simulink model "single_phase_afe_ideal"  (R2026a)
settings: Solver=ode23tb  StopTime=simlength  FixedStep=tc  MaxStep=glb_time.tc
values from neighbouring files (symbols this model uses):
  afe_ctrl = ctrl_afe_setup(glb_time.ts_afe, grid_emu.omega_grid_nom)    [init_model_legacy.m]
  frequency_set = 300    [init_model_legacy.m]
  glb_time = timing_setup(fpwm_afe, trgo_afe, fpwm_inv, trgo_inv, fpwm_single_phase_inv, trgo_single_phase_inv, fpwm_dab, trgo_dab,      fpwm_psfbc, trgo_psfbc, fpwm_isop_rail, trgo_isop_rail, fpwm_cllc, trgo_cllc, t_measure, tc_factor, tc_decimation, delay_pwm, dead_time_afe,      dead_time_inv, dead_time_single_phase_inv, dead_time_dab, dead_time_psfbc, dead_time_isop_rail, dead_time_cllc)    [init_model_legacy.m]
  grid_emu = grid_three_phase_emulator('Dyn11', delta_star, grid_nominal_power, application_voltage, us1, us2, fgrid,                  eq_grid_inductance, eq_grid_resistance, eta, ucc, i1m, p_iron, n1, n2, core_area, core_length, mur,                  up_xi_pu_ref, up_eta_pu_ref, un_xi_pu_ref, un_eta_pu_ref)    [init_model_legacy.m]
  heatsink = liquid_cooled_plate_2kw_setup(weight, no_weight, cp_al, heat_capacity_hs, thermal_conductivity_al,      Rth_switch_HA, Rth_mosfet_HA, Rth_diode_HA, Tambient, DThs_init)    [init_model_legacy.m]
  kepsilon = 2    [init_model_legacy.m]
  omega_set = frequency_set*2*pi    (= 1884.95559215)    [init_model_legacy.m]
  single_phase_inverter_ctrl = ctrl_single_phase_inverter_setup(glb_time.ts_inv, pres_ctrl.omega_set,      dqvector_pi.kp_inv, dqvector_pi.ki_inv, pres_ctrl.kp_rpi, pres_ctrl.ki_rpi, pres_ctrl.delta_rpi)    [init_model_legacy.m]
  Tambient = 40    [init_model_legacy.m]
  time_step_ref_1 = 0.025    [init_model_legacy.m]
  time_step_ref_2 = 0.5    [init_model_legacy.m]
  time_step_ref_3 = 1    [init_model_legacy.m]
  Vdc_nom = 400*1.35    (= 540)    [power_losses_calculation.m]
undefined symbols (not defined in the file or in its folder): delta_fht1, hwdata, igbt, Ld_fht1, magnitude, omega_fht1, ts_inv, Vac_FS, Xbez
libraries: fl_lib x116, nesl_utility x65, phase_shift_filter_ccaller x5, dq_vector_pi x4, igbt_simple_2th_lib x4, linear_double_integrator_observer_ccaller x3, lithium_ion_battery x1, dclink_for_two_levels x1, three_phase_voltage_with_frt_emulator x1, simulink x1, cstblocks_lti x1, single_phase_pwm_modulator x1
(part 6 of 6)

== matlab function single_phase_afe_ideal/single_phase_inverter/single phase inverter control/single_phase_inverter_ctrl/dclink_ripple_compensation_rpi/dq2alphabeta/MATLAB Function ==
  data: d input; alpha output; q input; phase input; beta output
function [alpha, beta] = dq2alphabeta(d, q, phase)

alpha = d*cos(phase) - q*sin(phase);
beta = d*sin(phase) + q*cos(phase);

== matlab function single_phase_afe_ideal/single_phase_inverter/single phase inverter control/single_phase_inverter_ctrl/phase generator/FHT-PLL/pll_stageB/double_integrator_observer/bounder2 ==
  data: u input; y output
function y = bounder(u)
    
    y = -pi + mod(u+3*pi,2*pi);
    
end

== matlab function single_phase_afe_ideal/single_phase_inverter/single phase inverter control/single_phase_inverter_ctrl/dclink_ripple_compensation_dq/dq_vector_pi1/alphabeta2dq/MATLAB Function ==
  data: alpha input; d output; beta input; phase input; q output
function [d, q] = alphabeta2dq(alpha, beta, phase)

d = alpha*cos(phase) + beta*sin(phase);
q = -alpha*sin(phase) + beta*cos(phase);

== matlab function single_phase_afe_ideal/single_phase_inverter/single phase inverter control/single_phase_inverter_ctrl/phase generator/FHT-PLL/pll_stageA/filter_and_transformation/abc2alphabeta ==
  data: a input; alpha output; b input; c input; beta output
function [alpha,beta] = abc2alphabeta(a,b,c)

alpha = 2/3*(a - 1/2*b - 1/2*c);
beta  = 1/sqrt(3)*(b - c);

end

== matlab function single_phase_afe_ideal/single_phase_inverter/single phase inverter control/single_phase_inverter_ctrl/dclink_ripple_compensation_dq/alphabeta2dq/MATLAB Function ==
  data: alpha input; d output; beta input; phase input; q output
function [d, q] = alphabeta2dq(alpha, beta, phase)

d = alpha*cos(phase) + beta*sin(phase);
q = -alpha*sin(phase) + beta*cos(phase);

== matlab function single_phase_afe_ideal/single_phase_inverter/single phase inverter control/single_phase_inverter_ctrl/phase generator/FHT-PLL/pll_stageA/sequences/alphabeta2xieta ==
  data: alpha input; xi output; beta input; gamma input; eta output
function [xi,eta] = alphabeta2xieta_pos(alpha,beta,gamma)

    xi  =  (alpha*cos(gamma) + beta*sin(gamma));
    eta = (-alpha*sin(gamma) + beta*cos(gamma));

end

== matlab function single_phase_afe_ideal/single_phase_inverter/single phase inverter control/single_phase_inverter_ctrl/sistem_identification/open loop u//f/dq2alphabeta/MATLAB Function ==
  data: d input; alpha output; q input; phase input; beta output
function [alpha, beta] = dq2alphabeta(d, q, phase)

alpha = d*cos(phase) - q*sin(phase);
beta = d*sin(phase) + q*cos(phase);

== matlab function single_phase_afe_ideal/single_phase_inverter/single phase inverter control/single_phase_inverter_ctrl/single_phase_current_control/dqpi_current_controller/alphabeta2dq/MATLAB Function ==
  data: alpha input; d output; beta input; phase input; q output
function [d, q] = alphabeta2dq(alpha, beta, phase)

d = alpha*cos(phase) + beta*sin(phase);
q = -alpha*sin(phase) + beta*cos(phase);

== matlab function single_phase_afe_ideal/single_phase_inverter/single phase inverter control/single_phase_inverter_ctrl/single_phase_current_control/dqpi_current_controller/dq2alphabeta/MATLAB Function ==
  data: d input; alpha output; q input; phase input; beta output
function [alpha, beta] = dq2alphabeta(d, q, phase)

alpha = d*cos(phase) - q*sin(phase);
beta = d*sin(phase) + q*cos(phase);
